simulink model "ASK"  (R2023b)
settings: Solver=VariableStepAuto  StartTime=0.0  StopTime=30  RelTol=1e-3
libraries: commrandsrc3 x1
settings Model: Creator=lxl  LastModifiedBy=lxl

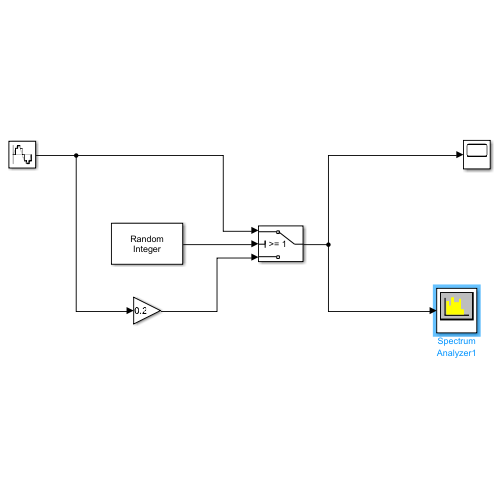
[thumbnail: Simulink's stored preview of the top-level diagram]
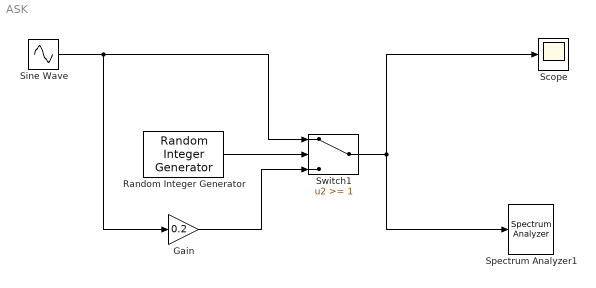
== system ASK ==
  Gain : Gain  Gain=0.2
  Random Integer Generator : commrandsrc3/Random Integer Generator  SetSize=2  SeedSource=Auto  Seed=0  SampleTime=0.5  SamplesPerFrame=1  OutputDataType=double  SimulateUsing=Interpreted execution
  Scope : Scope
  Sine Wave : Sin  Frequency=2*pi*10  SampleTime=1/100
  Spectrum Analyzer1 : SpectrumAnalyzer  WindowPosition=[368.000000,182.000000,800.000000,500.000000,]  ScopeFrameLocation=window  Span=100  StartFrequency=-50  StopFrequency=50  YLimits=[-165.57150698,-70.68978358]
  Switch1 : Switch  Threshold=1  SaturateOnIntegerOverflow=off  InputSameDT=off
  wires:
  Random Integer Generator/1 -> Switch1/2
  Gain/1 -> Switch1/3
  Switch1/1 -> Spectrum Analyzer1/1, Scope/1
  Sine Wave/1 -> Gain/1, Switch1/1
